simulink model "VFDnow"  (R2025b)
settings: Solver=VariableStepAuto  StartTime=0.0  StopTime=10  RelTol=1e-3
libraries: ee_lib x17, nesl_utility x12, fl_lib x10, dspstat3 x3, eePwmGeneratorTwoLevel x1, eeSinGeneratorThreePhase x1, simulink x1
settings Model: Creator=Administrator  LastModifiedBy=Nandana
settings SolverCC: AlgebraicLoopSolver=TrustRegion
settings DebuggingCC: UnconnectedInputMsg=warning  UnconnectedOutputMsg=warning  UnconnectedLineMsg=warning
settings ModelReferenceCC: EnableRefExpFcnMdlSchedulingChecks=on
settings SFSimCC: CustomCodeUndefinedFunction=UseInterfaceOnly
settings RTWCC: GPUComputeCapability=3.5  DLArmComputeVersion=19.05

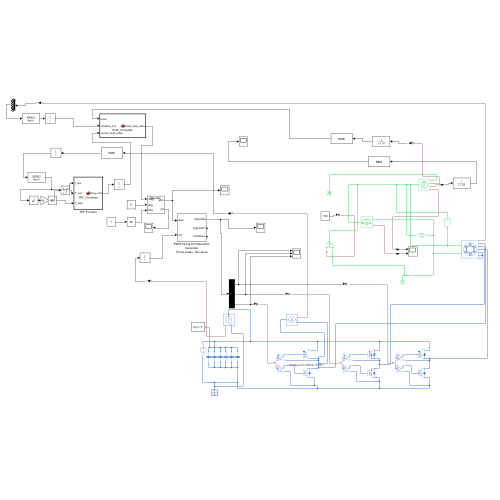
[thumbnail: Simulink's stored preview of the top-level diagram]
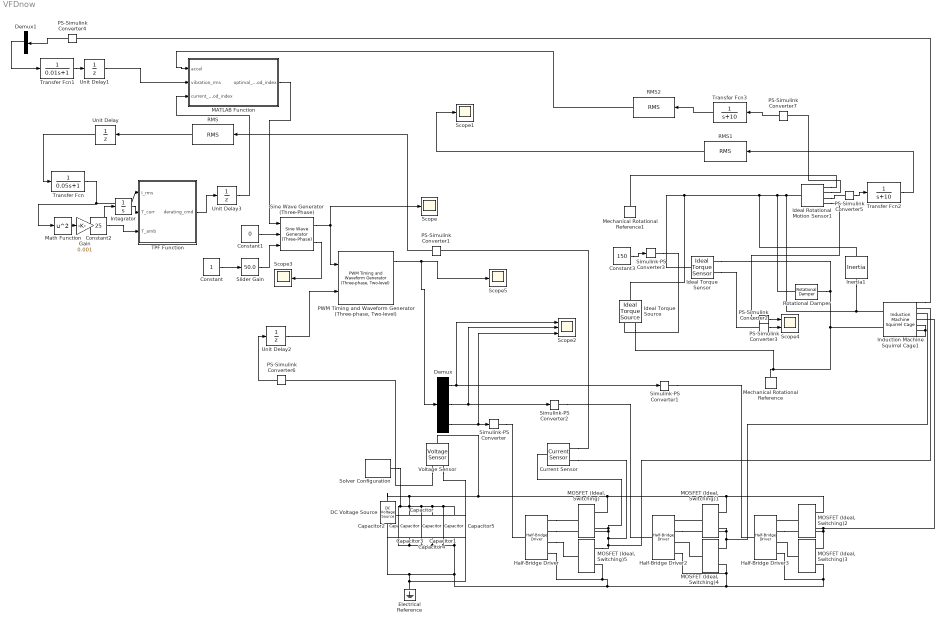
== system VFDnow ==
  Capacitor{,1..5} (6 alike) : ee_lib/Passive/Capacitor  cap_option=ee.enum.passive.capacitor.capOption.const  c=550e-6 F  Cvec=[1e-05, 1e-06] F  Vvec=[0, 10] V  CV_table_symmetry=ee.enum.passive.capacitor.tableSymmetry.yes  f_vec=[1, 10] kHz  DFext_vec=[.8, 1.2]  enable_C_tol=ee.enum.toleranceApplication.none  averaging_period=0 s  C_tol=5  tol_distribution=ee.enum.toleranceDistribution.uniform  nSigma=4  r=1 Ohm  g=0 1/Ohm  enable_operating_limits=ee.enum.enable.no  operating_limit_action=ee.enum.passive.reportOpLim.warn  max_working_voltage_range=[-25, 25] V  power_rating=1 W  maxTemperature=85 degC  thermalEnable=false  thermalMass=1 J/K  i_specify=off  i_priority=None  i=0 A  i_nominal_specify=off  i_nominal_value=1  i_nominal_unit=A  v_specify=on  v_priority=None  v=565 V  v_nominal_specify=off  v_nominal_value=1  v_nominal_unit=V  vc_specify=off  vc_priority=High  vc=0 V  vc_nominal_specify=off  vc_nominal_value=1  vc_nominal_unit=V  T_specify=off  T_priority=None  T=298.15 K  T_nominal_specify=off  T_nominal_value=1  T_nominal_unit=K
  Constant : Constant  SampleTime=1e-6
  Constant1 : Constant  Value=0  SampleTime=1e-6
  Constant2 : Constant  Value=25  SampleTime=1e-6
  Constant3 : Constant  Value=150  SampleTime=1e-6
  Current Sensor : fl_lib/Electrical/Electrical Sensors/Current Sensor
  DC Voltage Source : ee_lib/Additional Components/SPICE Sources/DC Voltage Source  DC=650 V
  Demux : Demux  Outputs=3
  Demux1 : Demux  Outputs=8
  Electrical Reference : fl_lib/Electrical/Electrical Elements/Electrical Reference
  Gain : Gain  Gain=0.001
  Half-Bridge Driver : ee_lib/Semiconductors & Converters/Half-Bridge Driver  port_option=ee.enum.controlport.ps  uHigh=2.0 V  uLow=0.8 V  uHighValue=0.7  uLowValue=0.3  vHigh=15 V  vLow=0 V  tpLH=50 ns  tdLH=100 ns  tpHL=50 ns  tdHL=100 ns  parameterization=ee.enum.semiconductors.gateDriverParam.outputImpedance  rHigh=2 Ohm  rLow=2 Ohm  tRise=20 ns  tFall=20 ns  cLoad=10 nF  ZonTime_specify=off  ZonTime_priority=None  ZonTime=0 s  ZoffTime_specify=off  ZoffTime_priority=None  ZoffTime=0 s  power_dissipated_high_side_specify=off  power_dissipated_high_side_priority=None  power_dissipated_high_side=0 W  power_dissipated_high_side_nominal_specify=off  power_dissipated_high_side_nominal_value=1  power_dissipated_high_side_nominal_unit=W  power_dissipated_low_side_specify=off  power_dissipated_low_side_priority=None  power_dissipated_low_side=0 W  power_dissipated_low_side_nominal_specify=off  power_dissipated_low_side_nominal_value=1  power_dissipated_low_side_nominal_unit=W
      settings: InternalSimscapePortConfiguration="{\"Bottom\":[],\"Left\":[{\"id\":\"u\",\"label\":\"u\",\"type\":\"input\"}],\"Right\":[{\"id\":\"HO\",\"label\":\"HO\",\"type\":\"foundation.electrical.electrical\"},{\"id\":\"HS\",\"label\":\"HS\",\"type\":\"foundation.electrical.electrical\"},{\"id\":\"LO\",\"label\":\"LO\",\"type\":\"foundation.electrical.electrical\"},{\"id\":\"LS\",\"label\":\"LS\",\"type\":\"foundation.electrical.electrical\"}],\"Top\":[]}"
  Half-Bridge Driver2 : ee_lib/Semiconductors & Converters/Half-Bridge Driver  port_option=ee.enum.controlport.ps  uHigh=2.0 V  uLow=0.8 V  uHighValue=0.7  uLowValue=0.3  vHigh=15 V  vLow=0 V  tpLH=50 ns  tdLH=100 ns  tpHL=50 ns  tdHL=100 ns  parameterization=ee.enum.semiconductors.gateDriverParam.outputImpedance  rHigh=2 Ohm  rLow=2 Ohm  tRise=20 ns  tFall=20 ns  cLoad=10 nF  ZonTime_specify=off  ZonTime_priority=None  ZonTime=0 s  ZoffTime_specify=off  ZoffTime_priority=None  ZoffTime=0 s  power_dissipated_high_side_specify=off  power_dissipated_high_side_priority=None  power_dissipated_high_side=0 W  power_dissipated_high_side_nominal_specify=off  power_dissipated_high_side_nominal_value=1  power_dissipated_high_side_nominal_unit=W  power_dissipated_low_side_specify=off  power_dissipated_low_side_priority=None  power_dissipated_low_side=0 W  power_dissipated_low_side_nominal_specify=off  power_dissipated_low_side_nominal_value=1  power_dissipated_low_side_nominal_unit=W
      settings: InternalSimscapePortConfiguration="{\"Bottom\":[],\"Left\":[{\"id\":\"u\",\"label\":\"u\",\"type\":\"input\"}],\"Right\":[{\"id\":\"HO\",\"label\":\"HO\",\"type\":\"foundation.electrical.electrical\"},{\"id\":\"HS\",\"label\":\"HS\",\"type\":\"foundation.electrical.electrical\"},{\"id\":\"LO\",\"label\":\"LO\",\"type\":\"foundation.electrical.electrical\"},{\"id\":\"LS\",\"label\":\"LS\",\"type\":\"foundation.electrical.electrical\"}],\"Top\":[]}"
  Half-Bridge Driver3 : ee_lib/Semiconductors & Converters/Half-Bridge Driver  port_option=ee.enum.controlport.ps  uHigh=2.0 V  uLow=0.8 V  uHighValue=0.7  uLowValue=0.3  vHigh=15 V  vLow=0 V  tpLH=50 ns  tdLH=100 ns  tpHL=50 ns  tdHL=100 ns  parameterization=ee.enum.semiconductors.gateDriverParam.outputImpedance  rHigh=2 Ohm  rLow=2 Ohm  tRise=20 ns  tFall=20 ns  cLoad=10 nF  ZonTime_specify=off  ZonTime_priority=None  ZonTime=0 s  ZoffTime_specify=off  ZoffTime_priority=None  ZoffTime=0 s  power_dissipated_high_side_specify=off  power_dissipated_high_side_priority=None  power_dissipated_high_side=0 W  power_dissipated_high_side_nominal_specify=off  power_dissipated_high_side_nominal_value=1  power_dissipated_high_side_nominal_unit=W  power_dissipated_low_side_specify=off  power_dissipated_low_side_priority=None  power_dissipated_low_side=0 W  power_dissipated_low_side_nominal_specify=off  power_dissipated_low_side_nominal_value=1  power_dissipated_low_side_nominal_unit=W
      settings: InternalSimscapePortConfiguration="{\"Bottom\":[],\"Left\":[{\"id\":\"u\",\"label\":\"u\",\"type\":\"input\"}],\"Right\":[{\"id\":\"HO\",\"label\":\"HO\",\"type\":\"foundation.electrical.electrical\"},{\"id\":\"HS\",\"label\":\"HS\",\"type\":\"foundation.electrical.electrical\"},{\"id\":\"LO\",\"label\":\"LO\",\"type\":\"foundation.electrical.electrical\"},{\"id\":\"LS\",\"label\":\"LS\",\"type\":\"foundation.electrical.electrical\"}],\"Top\":[]}"
  Ideal Rotational Motion Sensor1 : fl_lib/Mechanical/Mechanical Sensors/Ideal Rotational Motion Sensor  reference=foundation.enum.MeasurementReference.difference  acceleration_port=true  velocity_port=true  position_port=true  wrap_angle=false  offset=0 rad
      settings: InternalSimscapePortConfiguration="{\"Bottom\":[],\"Left\":[{\"id\":\"R\",\"label\":\"R\",\"type\":\"foundation.mechanical.rotational.rotational\"}],\"Right\":[{\"id\":\"C\",\"label\":\"C\",\"type\":\"foundation.mechanical.rotational.rotational\"},{\"id\":\"alpha\",\"label\":\"α\",\"type\":\"output\"},{\"id\":\"W\",\"label\":\"W\",\"type\":\"output\"},{\"id\":\"A\",\"label\":\"A\",\"type\":\"output\"}],\"Top\":[]}"
  Ideal Torque Sensor : fl_lib/Mechanical/Mechanical Sensors/Ideal Torque Sensor
  Ideal Torque Source : fl_lib/Mechanical/Mechanical Sources/Ideal Torque Source
  Induction Machine Squirrel Cage1 : ee_lib/Electromechanical/Asynchronous/Induction Machine Squirrel Cage  port_option=ee.enum.threePhasePort.expanded  SRated=15e3 A*V  VRated=220 V  FRated=60 Hz  nPolePairs=1  param_unit=ee.enum.unit.si  squirrel_cage=ee.enum.squirrelcage.Single  zero_sequence=ee.enum.park.zerosequence.include  initialization_option=ee.enum.asm.initialization.fluxvariables  Rs=0.25 Ohm  Xls=0.4 Ohm  pu_Rs=0.0258  pu_Lls=0.0413  Rrd=0.14 Ohm  Xlrd=0.41 Ohm  pu_Rrd=0.0145  pu_Llrd=0.0424  Rrd1=0.28 Ohm  Xlrd1=0.82 Ohm  Rrd2=0.28 Ohm  Xlrd2=0.82 Ohm  pu_Rrd1=0.0290  pu_Llrd1=0.0848  pu_Rrd2=0.0290  pu_Llrd2=0.0848  Xm=17 Ohm  pu_Lm=1.7562  X0=0.4 Ohm  pu_L0=0.0413  saturation_option=ee.enum.saturation.exclude  saturation_i=[0, 4, 9, 18, 25, 34, 50, 68, 95, 120] A  saturation_v=[0, 88, 154, 198, 220, 242, 264, 286, 308, 327] V  pu_saturation_i=[0, .176, .396, .792, 1.1, 1.496, 2.2, 2.992, 4.18, 5.28]  pu_saturation_v=[0, .4, .7, .9, 1, 1.1, 1.2, 1.3, 1.4, 1.4864]  connection_option=ee.enum.Connection.delta  angular_position_specify=off  angular_position_priority=None  angular_position=0 deg  angular_position_nominal_specify=off  angular_position_nominal_value=1  angular_position_nominal_unit=deg  pu_psids_specify=off  pu_psids_priority=None  pu_psids=0  pu_psids_nominal_specify=off  pu_psids_nominal_value=1  pu_psids_nominal_unit=1  pu_psiqs_specify=off  pu_psiqs_priority=None  pu_psiqs=0  pu_psiqs_nominal_specify=off  pu_psiqs_nominal_value=1  pu_psiqs_nominal_unit=1  pu_psi0s_specify=off  pu_psi0s_priority=None  pu_psi0s=0  pu_psi0s_nominal_specify=off  pu_psi0s_nominal_value=1  pu_psi0s_nominal_unit=1  pu_psidr_specify=off  pu_psidr_priority=None  pu_psidr=0  pu_psidr_nominal_specify=off  pu_psidr_nominal_value=1  pu_psidr_nominal_unit=1  pu_psiqr_specify=off  pu_psiqr_priority=None  pu_psiqr=0  pu_psiqr_nominal_specify=off  pu_psiqr_nominal_value=1  pu_psiqr_nominal_unit=1  pu_psidr1_specify=off  pu_psidr1_priority=None  pu_psidr1=0  pu_psidr1_nominal_specify=off  pu_psidr1_nominal_value=1  pu_psidr1_nominal_unit=1  pu_psiqr1_specify=off  pu_psiqr1_priority=None  pu_psiqr1=0  pu_psiqr1_nominal_specify=off  pu_psiqr1_nominal_value=1  pu_psiqr1_nominal_unit=1  pu_psidr2_specify=off  pu_psidr2_priority=None  pu_psidr2=0  pu_psidr2_nominal_specify=off  pu_psidr2_nominal_value=1  pu_psidr2_nominal_unit=1  pu_psiqr2_specify=off  pu_psiqr2_priority=None  pu_psiqr2=0  pu_psiqr2_nominal_specify=off  pu_psiqr2_nominal_value=1  pu_psiqr2_nominal_unit=1  psids_specify=off  psids_priority=None  psids=0 Wb  psids_nominal_specify=off  psids_nominal_value=1  psids_nominal_unit=Wb  psiqs_specify=off  psiqs_priority=None  psiqs=0 Wb  psiqs_nominal_specify=off  psiqs_nominal_value=1  psiqs_nominal_unit=Wb  psi0s_specify=off  psi0s_priority=None  psi0s=0 Wb  psi0s_nominal_specify=off  psi0s_nominal_value=1  psi0s_nominal_unit=Wb  psidr_specify=off  psidr_priority=None  psidr=0 Wb  psidr_nominal_specify=off  psidr_nominal_value=1  psidr_nominal_unit=Wb  psiqr_specify=off  psiqr_priority=None  psiqr=0 Wb  psiqr_nominal_specify=off  psiqr_nominal_value=1  psiqr_nominal_unit=Wb  psidr1_specify=off  psidr1_priority=None  psidr1=0 Wb  psidr1_nominal_specify=off  psidr1_nominal_value=1  psidr1_nominal_unit=Wb  psiqr1_specify=off  psiqr1_priority=None  psiqr1=0 Wb  psiqr1_nominal_specify=off  psiqr1_nominal_value=1  psiqr1_nominal_unit=Wb  psidr2_specify=off  psidr2_priority=None  psidr2=0 Wb  psidr2_nominal_specify=off  psidr2_nominal_value=1  psidr2_nominal_unit=Wb  psiqr2_specify=off  psiqr2_priority=None  psiqr2=0 Wb  psiqr2_nominal_specify=off  psiqr2_nominal_value=1  psiqr2_nominal_unit=Wb  slip_specify=off  slip_priority=None  slip=0  slip_nominal_specify=off  slip_nominal_value=1  slip_nominal_unit=1  real_power_generated_specify=off  real_power_generated_priority=None  real_power_generated=0 W  real_power_generated_nominal_specify=off  real_power_generated_nominal_value=1  real_power_generated_nominal_unit=W  mechanical_power_consumed_specify=off  mechanical_power_consumed_priority=None  mechanical_power_consumed=0 W  mechanical_power_consumed_nominal_specify=off  mechanical_power_consumed_nominal_value=1  mechanical_power_consumed_nominal_unit=W  Tmeas=298.15 K  alpha=3.93e-3 1/K  alpha_cage=4.4e-3 1/K  stator_thermal_mass=100 J/K  rotor_thermal_mass=200 J/K  temperatureA_specify=off  temperatureA_priority=High  temperatureA=25 degC  temperatureA_nominal_specify=off  temperatureA_nominal_value=1  temperatureA_nominal_unit=degC  temperatureB_specify=off  temperatureB_priority=High  temperatureB=25 degC  temperatureB_nominal_specify=off  temperatureB_nominal_value=1  temperatureB_nominal_unit=degC  temperatureC_specify=off  temperatureC_priority=High  temperatureC=25 degC  temperatureC_nominal_specify=off  temperatureC_nominal_value=1  temperatureC_nominal_unit=degC  temperatureR_specify=off  temperatureR_priority=High  temperatureR=25 degC  temperatureR_nominal_specify=off  temperatureR_nominal_value=1  temperatureR_nominal_unit=degC
      settings: InternalSimscapePortConfiguration="{\"Bottom\":[],\"Left\":[{\"id\":\"R\",\"label\":\"R\",\"type\":\"foundation.mechanical.rotational.rotational\"},{\"id\":\"C\",\"label\":\"C\",\"type\":\"foundation.mechanical.rotational.rotational\"}],\"Right\":[{\"id\":\"pu_output\",\"label\":\"pu\",\"type\":\"output\"},{\"id\":\"a1\",\"label\":\"a1\",\"type\":\"foundation.electrical.electrical\"},{\"id\":\"b1\",\"label\":\"b1\",\"type\":\"foundation.electrical.electrical\"},{\"id\":\"c1\",\"label\":\"c1\",\"type\":\"foundation.electrical.electrical\"},{\"id\":\"a2\",\"label\":\"a2\",\"type\":\"foundation.electrical.electrical\"},{\"id\":\"b2\",\"label\":\"b2\",\"type\":\"foundation.electrical.electrical\"},{\"id\":\"c2\",\"label\":\"c2\",\"type\":\"foundation.electrical.electrical\"}],\"Top\":[]}"
  Inertia1 : fl_lib/Mechanical/Rotational Elements/Inertia  inertia=1.8 kg*m^2  num_ports=foundation.enum.numPorts2.two  w_specify=off  w_priority=High  w=0 rad/s  w_nominal_specify=off  w_nominal_value=1  w_nominal_unit=rad/s  t_specify=off  t_priority=None  t=0 N*m  t_nominal_specify=off  t_nominal_value=1  t_nominal_unit=N*m
      settings: InternalSimscapePortConfiguration="{\"Bottom\":[],\"Left\":[{\"id\":\"I\",\"label\":\"\",\"type\":\"foundation.mechanical.rotational.rotational\"}],\"Right\":[{\"id\":\"J\",\"label\":\"\",\"type\":\"foundation.mechanical.rotational.rotational\"}],\"Top\":[]}"
  Integrator : Integrator  InitialCondition=25  LimitOutput=on  UpperSaturationLimit=100  LowerSaturationLimit=25
  MATLAB Function : MATLAB Function  TreatAsAtomicUnit=on
  "MOSFET (Ideal, Switching)" : ee_lib/Semiconductors & Converters/MOSFET (Ideal, Switching)  PartSpecification="{\"CollectionId\":\"SimscapeElectrical\",\"CollectionVersion\":\"1.0.0\",\"DatasetId\":\"Wolfspeed|C3M0021120K1|\",\"DisplayName\":\"Wolfspeed:C3M0021120K1\"}"  port_option=ee.enum.controlport.elec  Rds=0.021 % Datasheet derived Ohm  Goff=8.33333333333333e-10 % Datasheet derived S  Vth=2.9 % Wolfspeed XML derived V  diode_param=ee.enum.converters.protectiondiode.nodynamics  diode_Vf=2.47 % Datasheet derived V  diode_Ron=0.012 % Wolfspeed XML derived Ohm  diode_Goff=1e-05 % Library default S  diode_C=50e-9 % Parameter not set F  diode_iRM=-235 % Parameter not set A  diode_iF=300 % Parameter not set A  diode_idot=-50 % Parameter not set A/us  diode_trr_param=ee.enum.converters.diodeReverseParam.trr_factor  diode_trr_factor=3 % Parameter not set  diode_trr=15 % Parameter not set us  diode_Qrr=1500 % Parameter not set s*uA  ids_specify=on  ids_priority=None  ids=0 A  ids_nominal_specify=on  ids_nominal_value=1  ids_nominal_unit=A  vds_specify=on  vds_priority=None  vds=0 V  vds_nominal_specify=on  vds_nominal_value=1  vds_nominal_unit=V  vgs_specify=off  vgs_priority=None  vgs=0 V  vgs_nominal_specify=off  vgs_nominal_value=1  vgs_nominal_unit=V  thermal_loss_option=ee.enum.converters.thermalLossOption.tabulated2d  Von_data=[-4.27389 -4.02367 -3.77256 -3.51776 -3.26306 -3.00223 -2.73772 -2.46956 -2.19212 -1.90551 -1.60743 -1.29443 -0.962781 -0.606415 -0.31632 -0.214648 -0.108889 -0.0455276 -0.0237427 0 0.0228239 0.0433363 0.106503 0.214663 0.323026 0.662263 1.13841 1.64037 2.16245 2.70962 3.28471 3.8982 4.56044 5.2802 6.07016 6.93522;-5.18634 -4.76738 -4.4029 -4.06633 -3.72922 -3.39492 -3.05953 -2.72304 -2.38461 -2.04123 -1.69306 -1.33736 -0.97293 -0.595048 -0.302935 -0.206772 -0.104318 -0.0429045 -0.0221598 0 0.0232804 0.0430606 0.104009 0.206365 0.308279 0.6242 1.06384 1.5255 2.0111 2.52481 3.07168 3.65807 4.29107 4.98079 5.73956 6.58181;-8.32654 -7.93499 -7.51349 -7.06183 -6.57553 -6.05033 -5.48279 -4.87921 -4.25441 -3.61939 -2.97325 -2.32248 -1.66914 -1.01052 -0.510784 -0.341428 -0.172389 -0.0707504 -0.0361764 0 0.0365721 0.0707068 0.173457 0.346572 0.520136 1.04549 1.76862 2.5225 3.31582 4.16389 5.07499 6.06793 7.16531 8.3916 9.78437 11.3885;-9.1592 -8.72849 -8.26484 -7.76802 -7.23309 -6.65536 -6.03107 -5.36713 -4.67985 -3.98133 -3.27058 -2.55473 -1.83605 -1.11158 -0.561862 -0.375571 -0.189628 -0.0778255 -0.039794 0 0.0402293 0.0777775 0.190803 0.381229 0.57215 1.15004 1.94548 2.77475 3.6474 4.58028 5.58249 6.67472 7.88184 9.23076 10.7628 12.5274] % Wolfspeed XML derived V  Tj=[-55 25 175 900] % Wolfspeed XML derived degC  Iout_data=[-290 -270 -250 -230 -210 -190 -170 -150 -130 -110 -90 -70 -50 -30 -15 -10 -5 -2 -1 0 1 2 5 10 15 30 50 70 90 110 130 150 170 190 210 230] % Wolfspeed XML derived A  Eon_data=[0 0.00041745 0.0006665 0.0009583 0.0013038 0.0016836 0.0021011 0.0025367 0.0029961;0 0.00043908 0.00072163 0.0010599 0.001457 0.0018976 0.0023654 0.0028532 0.0033508;0 0.00049099 0.00084535 0.0012573 0.0017203 0.0022304 0.0027638 0.0032706 0.0036897;0 0.0005622 0.00099378 0.0014717 0.0019935 0.0025368 0.0030168 0.0033994 0.0036872;0 0.00061842 0.0010932 0.0016189 0.0021929 0.0027904 0.0033184 0.0037393 0.0040559] % Wolfspeed XML derived J  Eoff_data=[0 7.5223e-05 0.00013186 0.0002269 0.00034998 0.00048869 0.00064891 0.00082419 0.0010195;0 8.254e-05 0.000147 0.00025079 0.00037991 0.00052991 0.00069891 0.00088752 0.0010918;0 7.4201e-05 0.00015201 0.00026409 0.0004049 0.00056157 0.00074296 0.00093905 0.0011553;0 8.0776e-05 0.00015818 0.00028047 0.0004289 0.00059195 0.00078795 0.00099015 0.0012074;0 8.8853e-05 0.000174 0.00030852 0.00047179 0.00065115 0.00086674 0.0010892 0.0013281] % Wolfspeed XML derived J  Eon_data_3D=reshape([0;0;0;0;0;0;0;0;0;0;0;0;0;0;0;0;0;0;0;0;0;0;0;0;0;0;0;0;0;0;0;0;0;0;0;0;0;0;0;0;0;0;0;0;0;0;0;0;0;0;0;0;0;0;0;0;0;0;0;0;0;0;0;0;0;0;0;0;0;0;0;0;0;0;0;0;0;0;0;0;0;0;0;0;0;0;0;0;0;0;0;0;0;0;0;0.0002788;0.0002932;0.00032775;0.00037518;0.0004127;0.00043572;0.00047148;0.00055198;0.00064879;0.00071367;0.0006243;0.0006901;0.00081857;0.00095848;0.0010543;0.00085437;0.00095468;0.0011272;0.0013064;0.0014371;0.0010984;0.0012379;0.0014553;0.0016574;0.0018231;0.0013696;0.0015419;0.0018028;0.0019726;0.0021698;0.0016665;0.0018748;0.0021525;0.0022422;0.0024665;0.0019653;0.0021993;0.0024309;0.0024363;0.0026799;0;0;0;0;0;0.00041745;0.00043908;0.00049099;0.0005622;0.00061842;0.0006665;0.00072163;0.00084535;0.00099378;0.0010932;0.0009583;0.0010599;0.0012573;0.0014717;0.0016189;0.0013038;0.001457;0.0017203;0.0019935;0.0021929;0.0016836;0.0018976;0.0022304;0.0025368;0.0027904;0.0021011;0.0023654;0.0027638;0.0030168;0.0033184;0.0025367;0.0028532;0.0032706;0.0033994;0.0037393;0.0029961;0.0033508;0.0036897;0.0036872;0.0040559],[5 9 4]) % Wolfspeed XML derived J  Eoff_data_3D=reshape([0;0;0;0;0;0;0;0;0;0;0;0;0;0;0;0;0;0;0;0;0;0;0;0;0;0;0;0;0;0;0;0;0;0;0;0;0;0;0;0;0;0;0;0;0;0;0;0;0;0;0;0;0;0;0;0;0;0;0;0;0;0;0;0;0;0;0;0;0;0;0;0;0;0;0;0;0;0;0;0;0;0;0;0;0;0;0;0;0;0;0;0;0;0;0;4.6339e-05;5.0834e-05;4.5637e-05;4.9715e-05;5.4686e-05;8.9796e-05;0.00010011;0.00010338;0.00010758;0.00011833;0.00015204;0.00016814;0.00017697;0.00018789;0.00020668;0.00024257;0.00026333;0.00028065;0.0002973;0.00032703;0.00034178;0.00037067;0.00039283;0.00041406;0.00045547;0.00045429;0.00048937;0.00052024;0.00055174;0.00060691;0.0005861;0.00063122;0.00066795;0.00070456;0.00077502;0.00072968;0.00078189;0.00082724;0.00086523;0.00095175;0;0;0;0;0;7.5223e-05;8.254e-05;7.4201e-05;8.0776e-05;8.8853e-05;0.00013186;0.000147;0.00015201;0.00015818;0.000174;0.0002269;0.00025079;0.00026409;0.00028047;0.00030852;0.00034998;0.00037991;0.0004049;0.0004289;0.00047179;0.00048869;0.00052991;0.00056157;0.00059195;0.00065115;0.00064891;0.00069891;0.00074296;0.00078795;0.00086674;0.00082419;0.00088752;0.00093905;0.00099015;0.0010892;0.0010195;0.0010918;0.0011553;0.0012074;0.0013281],[5 9 4]) % Wolfspeed XML derived J  Tj_loss=[25 75 125 175 900] % Wolfspeed XML derived degC  Iout_data_loss=[0 16.48625 31.86563 46.89437 62.43531 76.75938 91.2175 105.2391 119.1231] % Wolfspeed XML derived A  tabulateWithVds=true  Vds_loss=[-100 0 600 800] % Wolfspeed XML derived V  Eon_scalar=22.86e-3 % Parameter not set J  Eoff_scalar=17.14e-3 % Parameter not set J  Voff=300 % Parameter not set V  Iout_scalar=600 % Parameter not set A  useCurrentFromPreviousCycle=false % Parameter not set  useVoltageFromPreviousCycle=false % Parameter not set  diodeModelType=ee.enum.converters.diodeModelType.tabulated  diodeTableType=ee.enum.diode.tableType.VfMat  diode_ReverseIVType=ee.enum.diode.diodeReverseIV.constant  diode_IfMat=[.07, .12, .19, 1.75, 4.24, 7.32, 11.2; .16, .3, .72, 2.14, 4.02, 6.35, 9.12] % Parameter not set A  diode_VfMat=[0 3.4539 3.7122 4.1778 4.6574 5.0077 5.7507 6.4353 6.9636 7.4039 7.7872 8.1335 8.4486 8.7404 9.0146 9.2743 9.5227 9.7598 9.9906;0 3.0632 3.2597 3.6226 4.0058 4.2921 4.9319 5.5601 6.0709 6.512 6.909 7.2724 7.6085 7.9244 8.2241 8.5101 8.7827 9.0425 9.2923;0 2.6447 2.8328 3.1828 3.5428 3.8081 4.3889 4.9604 5.4274 5.8323 6.1991 6.5353 6.8489 7.1419 7.4196 7.6847 7.9366 8.1816 8.4159;0 2.1158 2.2663 2.5462 2.8343 3.0464 3.5111 3.9683 4.3419 4.6658 4.9593 5.2283 5.4792 5.7135 5.9357 6.1478 6.3493 6.5453 6.7327] % Wolfspeed XML derived V  diode_TjVec=[-55 25 175 900] % Wolfspeed XML derived degC  diode_VfVec=[.5, .7, .9, 1.3, 1.7, 2.1, 2.5] % Parameter not set V  diode_IfVec=[0 1 2 5 10 15 30 50 70 90 110 130 150 170 190 210 230 250 270] % Wolfspeed XML derived A  diode_IrMat=[1e-06, 2e-06, 5e-06, 1e-05, 2.5e-05, 5e-05, .0001; 2e-06, 5e-06, 1e-05, 4e-05, 8e-05, .0002, .0005] % Parameter not set A  diode_VrMat=[10, 100, 200, 250, 300, 325, 350; 10, 70, 160, 220, 270, 300, 320] % Parameter not set V  diode_VrVec=[10, 20, 40, 50, 70, 80, 100] % Parameter not set V  diode_IrVec=[1e-06, 2e-06, 5e-06, 1e-05, 2e-05, 5e-05, .0001] % Parameter not set A  diode_Vr=-600 % Parameter not set V  diode_Ls=150 % Parameter not set nH  diode_Erec=0.03 % Parameter not set J  diode_rec_loss_model=ee.enum.diode.reverseRecoveryModel.tabulated2d  diode_ErecVal=0 % Parameter not set J  diode_scaleWithIandV=true % Parameter not set  diode_ErecMat=[0 0;0 0] % Wolfspeed XML derived J  diode_TjrecVec=[25 35] % Wolfspeed XML derived degC  diode_IfrecVec=[0 10] % Wolfspeed XML derived A  diode_IrecVal=10 % Parameter not set A  diode_VrecVal=10 % Wolfspeed XML derived V  diode_tFilter=1 / 1000 / 100 % Parameter not set s  separateThermalPortForDiode=true  thermal_network_parameterization=ee.enum.thermalNetworkTopology.cauer  Rth=[.03, .2] % Parameter not set K/W  Rth_Cauer=[0.040655 0.093503 0.046885 0.094584] % Wolfspeed XML derived K/W  Rth_Foster=[.08, .14, .22, .16] % Parameter not set K/W  thermal_mass_parameterization=ee.enum.thermalNetwork.thermalmass  thermal_mass=[3, 25] % Parameter not set J/K  thermal_mass_Cauer=[0.0029508 0.016009 0.049724 0.13401] % Wolfspeed XML derived J/K  thermal_mass_Foster=[.001, .005, .05, .5] % Parameter not set J/K  thermal_time_constant=[.1, 5] % Parameter not set s  thermal_time_constant_Cauer=[.1, 1, 5] % Parameter not set s  thermal_time_constant_Foster=[7e-05, .0007, .01, .08] % Parameter not set s  thermal_mass_initial_temperatures=[25, 25] % Parameter not set degC  thermal_mass_initial_temperatures_Cauer=[25 25 25 25] % Wolfspeed XML derived degC  junction_thermal_mass=0.1 % Parameter not set J/K  Tvec_initial_Foster=[25, 25, 25, 25] % Parameter not set degC  RthDiode=[.03, .2] % Parameter not set K/W  RthCauerDiode=[0.040655 0.093503 0.046885 0.094584] % Wolfspeed XML derived K/W  RthFosterDiode=[.03, .2] % Parameter not set K/W  thermalMassDiode=[3, 25] % Parameter not set J/K  thermalMassCauerDiode=[0.0029508 0.016009 0.049724 0.13401] % Wolfspeed XML derived J/K  thermalMassFosterDiode=[33, 50] % Parameter not set J/K  thermalTauDiode=[.1, 5] % Parameter not set s  thermalTauCauerDiode=[.1, 1, 5] % Parameter not set s  thermalTauFosterDiode=[1, 10] % Parameter not set s  thermalMassInitTempDiode=[25, 25] % Parameter not set degC  thermalMassInitTempCauerDiode=[25 25 25 25] % Wolfspeed XML derived degC  junctionthermalMassDiode=0.1 % Parameter not set J/K  TVecInitialFosterDiode=[25, 25, 25, 25] % Parameter not set degC  no_thermal_network=0 % Parameter not set  mosfet_junction_temperature_specify=off  mosfet_junction_temperature_priority=None  mosfet_junction_temperature=25 degC  mosfet_junction_temperature_nominal_specify=off  mosfet_junction_temperature_nominal_value=1  mosfet_junction_temperature_nominal_unit=degC  diode_junction_temperature_specify=off  diode_junction_temperature_priority=None  diode_junction_temperature=25 degC  diode_junction_temperature_nominal_specify=off  diode_junction_temperature_nominal_value=1  diode_junction_temperature_nominal_unit=degC  Qj_specify=off  Qj_priority=None  Qj=0 W  Qj_nominal_specify=off  Qj_nominal_value=1  Qj_nominal_unit=W  accumulatedSwitchingLosses_specify=off  accumulatedSwitchingLosses_priority=None  accumulatedSwitchingLosses=0 J
      settings: AttributesFormatString=Wolfspeed:C3M0021120K1  InternalSimscapePortConfiguration="{\"Bottom\":[],\"Left\":[{\"id\":\"G_elec\",\"label\":\"\",\"type\":\"foundation.electrical.electrical\"}],\"Right\":[{\"id\":\"D\",\"label\":\"\",\"type\":\"foundation.electrical.electrical\"},{\"id\":\"S\",\"label\":\"\",\"type\":\"foundation.electrical.electrical\"}],\"Top\":[]}"
  MOSFET (Ideal, Switching){1..5} (5 alike) : ee_lib/Semiconductors & Converters/MOSFET (Ideal, Switching)  port_option=ee.enum.controlport.elec  Rds=0.01 Ohm  Goff=1e-6 1/Ohm  Vth=2 V  diode_param=ee.enum.semiconductors.protectionDiode.nodynamics  diode_Vf=0.8 V  diode_Ron=0.001 Ohm  diode_Goff=1e-5 1/Ohm  diode_C=50e-9 F  diode_iRM=-235 A  diode_iF=300 A  diode_idot=-50 A/us  diode_trr_param=ee.enum.converters.diodeReverseParam.trr_factor  diode_trr_factor=3  diode_trr=15 us  diode_Qrr=1500 s*uA  ids_specify=off  ids_priority=None  ids=0 A  ids_nominal_specify=off  ids_nominal_value=1  ids_nominal_unit=A  vds_specify=off  vds_priority=None  vds=0 V  vds_nominal_specify=off  vds_nominal_value=1  vds_nominal_unit=V  vgs_specify=off  vgs_priority=None  vgs=0 V  vgs_nominal_specify=off  vgs_nominal_value=1  vgs_nominal_unit=V  thermal_loss_option=ee.enum.converters.thermalLossOption.constantvalues  Von_data=[0, 1.8, 3.2, 6, 10, 16; 0, 2, 5.5, 9.5, 15, 25] V  Tj=[298.15, 448.15] K  Iout_data=[0, 20, 40, 60, 80, 100] A  Eon_data=[0, 55.04, 124.57, 235.53, 362.12; 0, 71.25, 161.25, 304.88, 468.75] * 1e-6 J  Eoff_data=[0, 18, 30, 56.1, 76.5; 0, 22.5, 37.5, 70.13, 95.63] * 1e-6 J  Eon_data_3D=[zeros(2, 5, 3)] J  Eoff_data_3D=[zeros(2, 5, 3)] J  Tj_loss=[298.15, 448.15] K  Iout_data_loss=[0, 10, 20, 30, 40] A  tabulateWithVds=false  Vds_loss=[0, 150, 300] V  Eon_scalar=22.86e-3 J  Eoff_scalar=17.14e-3 J  Voff=300 V  Iout_scalar=600 A  useCurrentFromPreviousCycle=false  useVoltageFromPreviousCycle=false  diodeModelType=ee.enum.converters.diodeModelType.pwl  diodeTableType=ee.enum.diode.tableType.IfMat  diode_ReverseIVType=ee.enum.diode.diodeReverseIV.constant  diode_IfMat=[.07, .12, .19, 1.75, 4.24, 7.32, 11.2; .16, .3, .72, 2.14, 4.02, 6.35, 9.12] A  diode_VfMat=[.9, 1.15, 1.25, 1.5, 1.75, 2.17, 2.6, 2.85; .58, .68, .75, 1.1, 1.38, 1.77, 2.27, 2.7] V  diode_TjVec=[25, 125] degC  diode_VfVec=[.5, .7, .9, 1.3, 1.7, 2.1, 2.5] V  diode_IfVec=[.1, .2, .5, 1, 2, 4, 7, 10] A  diode_IrMat=[1e-06, 2e-06, 5e-06, 1e-05, 2.5e-05, 5e-05, .0001; 2e-06, 5e-06, 1e-05, 4e-05, 8e-05, .0002, .0005] A  diode_VrMat=[10, 100, 200, 250, 300, 325, 350; 10, 70, 160, 220, 270, 300, 320] V  diode_VrVec=[10, 20, 40, 50, 70, 80, 100] V  diode_IrVec=[1e-06, 2e-06, 5e-06, 1e-05, 2e-05, 5e-05, .0001] A  diode_Vr=-600 V  diode_Ls=150 nH  diode_Erec=0.03 J  diode_rec_loss_model=ee.enum.diode.reverseRecoveryModel.fixed  diode_ErecVal=0 J  diode_scaleWithIandV=true  diode_ErecMat=zeros(2, 3) J  diode_TjrecVec=[298.15, 398.15] K  diode_IfrecVec=[.1, 1, 10] A  diode_IrecVal=10 A  diode_VrecVal=10 V  diode_tFilter=1 / 1000 / 100 s  separateThermalPortForDiode=false  thermal_network_parameterization=ee.enum.thermalNetworkTopology.external  Rth=[.03, .2] K/W  Rth_Cauer=[.03, .1, .2] K/W  Rth_Foster=[.08, .14, .22, .16] K/W  thermal_mass_parameterization=ee.enum.thermalNetwork.timeconstant  thermal_mass=[3, 25] J/K  thermal_mass_Cauer=[3, 10, 25] J/K  thermal_mass_Foster=[.001, .005, .05, .5] J/K  thermal_time_constant=[.1, 5] s  thermal_time_constant_Cauer=[.1, 1, 5] s  thermal_time_constant_Foster=[7e-05, .0007, .01, .08] s  thermal_mass_initial_temperatures=[25, 25] degC  thermal_mass_initial_temperatures_Cauer=[25, 25, 25] degC  junction_thermal_mass=0.1 J/K  Tvec_initial_Foster=[25, 25, 25, 25] degC  RthDiode=[.03, .2] K/W  RthCauerDiode=[.03, .1, .2] K/W  RthFosterDiode=[.03, .2] K/W  thermalMassDiode=[3, 25] J/K  thermalMassCauerDiode=[3, 10, 25] J/K  thermalMassFosterDiode=[33, 50] J/K  thermalTauDiode=[.1, 5] s  thermalTauCauerDiode=[.1, 1, 5] s  thermalTauFosterDiode=[1, 10] s  thermalMassInitTempDiode=[25, 25] degC  thermalMassInitTempCauerDiode=[25, 25, 25] degC  junctionthermalMassDiode=0.1 J/K  TVecInitialFosterDiode=[25, 25, 25, 25] degC  no_thermal_network=0  mosfet_junction_temperature_specify=off  mosfet_junction_temperature_priority=None  mosfet_junction_temperature=25 degC  mosfet_junction_temperature_nominal_specify=off  mosfet_junction_temperature_nominal_value=1  mosfet_junction_temperature_nominal_unit=degC  diode_junction_temperature_specify=off  diode_junction_temperature_priority=None  diode_junction_temperature=25 degC  diode_junction_temperature_nominal_specify=off  diode_junction_temperature_nominal_value=1  diode_junction_temperature_nominal_unit=degC  Qj_specify=off  Qj_priority=None  Qj=0 W  Qj_nominal_specify=off  Qj_nominal_value=1  Qj_nominal_unit=W  accumulatedSwitchingLosses_specify=off  accumulatedSwitchingLosses_priority=None  accumulatedSwitchingLosses=0 J
      settings: InternalSimscapePortConfiguration="{\"Bottom\":[],\"Left\":[{\"id\":\"G_elec\",\"label\":\"\",\"type\":\"foundation.electrical.electrical\"}],\"Right\":[{\"id\":\"D\",\"label\":\"\",\"type\":\"foundation.electrical.electrical\"},{\"id\":\"S\",\"label\":\"\",\"type\":\"foundation.electrical.electrical\"}],\"Top\":[]}"
  Math Function : Math  Operator=square
  Mechanical Rotational Reference : fl_lib/Mechanical/Rotational Elements/Mechanical Rotational Reference
  Mechanical Rotational Reference1 : fl_lib/Mechanical/Rotational Elements/Mechanical Rotational Reference
  PS-Simulink Converter{1..2,4..7} (6 alike) : nesl_utility/PS-Simulink Converter  PhysicalDomain=network_engine_domain  SubClassName=ps_output  LeftPortType=input  RightPortType=output  PseudoPeriodic=off  Frequencies=[]  VectorFormat=inherit  Unit=inherit  AffineConversion=off
  PS-Simulink Converter3 : nesl_utility/PS-Simulink Converter  PhysicalDomain=network_engine_domain  SubClassName=ps_output  LeftPortType=input  RightPortType=output  PseudoPeriodic=off  Frequencies=[]  VectorFormat=inherit  Unit=rad  AffineConversion=off
  "PWM Timing and Waveform Generator (Three-phase, Two-level)" : eePwmGeneratorTwoLevel/PWM Timing and Waveform Generator (Three-phase, Two-level)  PWMMode=Continuous PWM (CPWM)  CPWMMode=SVM: space vector modulation  DPWMMode=60 DPWM (-30 degree shift): -30 degree shift from 60 DPWM  fsw=16000
      settings: SamplingMode=Natural
      settings: LibrarySourceBlock=|
      | ee_sl_lib/Pulse Width
      | Modulation/PWM Timing and Waveform
      | Generator
      | (Three-phase, Two-level)
  RMS : dspstat3/RMS  run=off  directionMode=Each column  dimension=1  InputProcessing=Columns as channels (frame based)  reset_popup=None
  RMS1 : dspstat3/RMS  run=off  directionMode=Each column  dimension=1  InputProcessing=Columns as channels (frame based)  reset_popup=None
  RMS2 : dspstat3/RMS  run=off  directionMode=Each column  dimension=1  InputProcessing=Columns as channels (frame based)  reset_popup=None
  Rotational Damper : fl_lib/Mechanical/Rotational Elements/Rotational Damper  D=0.05 N*m*s/rad  w_specify=off  w_priority=None  w=0 rad/s  w_nominal_specify=off  w_nominal_value=1  w_nominal_unit=rad/s  t_specify=off  t_priority=None  t=0 N*m  t_nominal_specify=off  t_nominal_value=1  t_nominal_unit=N*m
  Scope{,1,3,5} (4 alike) : Scope
      Scope settings: ActiveDisplayYMinimum=0.23817088996397734  ActiveDisplayYMaximum=0.25157848250419529
      Scope1 settings: ActiveDisplayYMinimum=-0.67417374525442053  ActiveDisplayYMaximum=1.0049836678211534
      Scope3 settings: ActiveDisplayYMinimum=-4.58577338507015  ActiveDisplayYMaximum=9.4544203181019419  DataLoggingVariableName=ScopeData3
      Scope5 settings: ActiveDisplayYMinimum=1.5573475654601123E-5  ActiveDisplayYMaximum=1.5676524345398877E-5  DataLoggingVariableName=ScopeData5
  Scope2 : Scope  NumInputPorts=3
      settings: ActiveDisplayYMinimum=1.559590351857362E-5  ActiveDisplayYMaximum=1.5647242039954659E-5  DataLoggingVariableName=ScopeData2
  Scope4 : Scope  NumInputPorts=2
      settings: ActiveDisplayYMinimum=-194.35610889768091  ActiveDisplayYMaximum=175.71484209304583  DataLoggingVariableName=ScopeData4
  Simulink-PS Converter{,1..3} (4 alike) : nesl_utility/Simulink-PS Converter  PhysicalDomain=network_engine_domain  SubClassName=ps_input  LeftPortType=input  RightPortType=output  PseudoPeriodic=off  Frequencies=[]  NoiseDistribution=none  NoiseParameters=[]  Unit=1  AffineConversion=off  FilteringAndDerivatives=provide  SimscapeFilterOrder=1  InputFilterTimeConstant=0.001  UdotUserProvided=0
  Sine Wave Generator (Three-Phase) : eeSinGeneratorThreePhase/Sine Wave Generator (Three-Phase)  Ts=1e-6
      settings: LibrarySourceBlock=|
      | ee_sl_lib/General Control/Sine Wave Generator
      | (Three-Phase)
  Slider Gain : simulink/Math Operations/Slider Gain  gain=50.0  low=0  high=100
  Solver Configuration : nesl_utility/Solver Configuration  PhysicalDomain=network_engine_domain  SubClassName=solver  LeftPortType=input  RightPortType=generic  Tones=[]  Harmonics=[]  SimulateNoise=off  Profile=off  UseLocalSampling=off  EnableSwitchedLinearOptims=on  FrequencyDomain=off  UseCCode=off  RelTol=0.001  AbsTol=0.001  MinStep=1e-09  ToWorkspace=off  RevertToSquareIcSolve=off  NumHomotopyIterations=100  PhasorMode=off  PhasorModeNumHarmonics=1  ConsistencySolver=NEWTON_XTOL_AFTER_FTOL  IndexReductionMethod=DerivativeReplacement  DoDC=off  ResidualTolerance=1e-09  ConsistencyTolSource=GLOBAL  ConsistencyAbsTol=0.001  ConsistencyRelTol=0.001  ConsistencyTolFactor=0.01  UseLocalSolver=on  LocalSolverChoice=NE_BACKWARD_EULER_ADVANCER  ResolveIndetEquations=on  FunctionEvalNumThread=1  LocalSolverSampleTime=1e-6  DoFixedCost=off  MaxNonlinIter=3  MaxModeIter=2  ComputeImpulses=off  ImpulseIterations=2  LinearAlgebra=Sparse  LinearAlgebraNumThread=0  EquationFormulation=NE_TIME_EF  DelaysMemoryBudget=1024  AutomaticFiltering=on  FilteringTimeConstant=0.001  PartitionStorageMethod=AS_NEEDED  PartitionMemoryBudget=1024  PartitionMethod=ROBUST  MultibodyUseLocalSolver=off  MultibodyLocalSolverChoice=ODE1  MultibodyLocalSolverSampleTime=0.001
  TPF Function : MATLAB Function  TreatAsAtomicUnit=on
  Transfer Fcn : TransferFcn  Denominator=[0.05 1]
  Transfer Fcn1 : TransferFcn  Denominator=[0.01 1]
  Transfer Fcn2 : TransferFcn  Denominator=[1 10]
  Transfer Fcn3 : TransferFcn  Denominator=[1 10]
  Unit Delay : UnitDelay  SampleTime=1e-6  HasFrameUpgradeWarning=on
  Unit Delay1 : UnitDelay  SampleTime=1e-6  HasFrameUpgradeWarning=on
  Unit Delay2 : UnitDelay  InitialCondition=600  SampleTime=1e-6  HasFrameUpgradeWarning=on
  Unit Delay3 : UnitDelay  SampleTime=1e-6  HasFrameUpgradeWarning=on
  Voltage Sensor : fl_lib/Electrical/Electrical Sensors/Voltage Sensor
  wires:
  Unit Delay2/1 -> "PWM Timing and Waveform Generator (Three-phase, Two-level)"/2
  PS-Simulink Converter6/1 -> Unit Delay2/1
  MATLAB Function/1(optimal_mod_index) -> Sine Wave Generator (Three-Phase)/1
  PS-Simulink Converter4/1 -> Demux1/1
  Unit Delay/1 -> Transfer Fcn/1
  Demux1/4 -> Transfer Fcn1/1
  RMS/1 -> Unit Delay/1
  Constant/1 -> Slider Gain/1
  Constant2/1 -> TPF Function/3(T_amb)
  Demux/2 -> Scope2/2, Simulink-PS Converter2/1
  Slider Gain/1 -> Sine Wave Generator (Three-Phase)/3
  Transfer Fcn/1 -> Math Function/1, TPF Function/1(I_rms)
  Demux/3 -> Scope2/3, Simulink-PS Converter/1
  Transfer Fcn1/1 -> Unit Delay1/1
  Math Function/1 -> Gain/1
  PS-Simulink Converter1/1 -> RMS/1
  Sine Wave Generator (Three-Phase)/2 -> Scope3/1
  Sine Wave Generator (Three-Phase)/1 -> "PWM Timing and Waveform Generator (Three-phase, Two-level)"/1, Scope/1
  Demux/1 -> Scope2/1, Simulink-PS Converter1/1
  Constant1/1 -> Sine Wave Generator (Three-Phase)/2
  Gain/1 -> Integrator/1
  Integrator/1 -> TPF Function/2(T_curr)
  TPF Function/1(derating_cmd) -> Unit Delay3/1
  Unit Delay3/1 -> MATLAB Function/3(current_mod_index)
  Constant3/1 -> Simulink-PS Converter3/1
  PS-Simulink Converter2/1 -> Scope4/2
  PS-Simulink Converter3/1 -> Scope4/1
  PS-Simulink Converter7/1 -> Transfer Fcn3/1
  Transfer Fcn3/1 -> RMS2/1
  PS-Simulink Converter5/1 -> Transfer Fcn2/1
  Transfer Fcn2/1 -> RMS1/1
  RMS1/1 -> Scope1/1
  RMS2/1 -> MATLAB Function/1(accel)
  "PWM Timing and Waveform Generator (Three-phase, Two-level)"/1 -> Scope5/1, Demux/1
  Unit Delay1/1 -> MATLAB Function/2(vibration_rms)
  connections:
  Half-Bridge Driver/RConn2 -- Current Sensor/LConn1 -- "MOSFET (Ideal, Switching)"/RConn2 -- Current Sensor/RConn2 -- "MOSFET (Ideal, Switching)5"/RConn1 -- Induction Machine Squirrel Cage1/RConn2
  DC Voltage Source/LConn1 -- Voltage Sensor/LConn1 -- "MOSFET (Ideal, Switching)2"/RConn1 -- "MOSFET (Ideal, Switching)1"/RConn1 -- "MOSFET (Ideal, Switching)"/RConn1 -- Solver Configuration/RConn1 -- Capacitor2/LConn1 -- Capacitor5/LConn1 -- Capacitor1/LConn1 -- Capacitor4/LConn1 -- Capacitor/LConn1 -- Capacitor3/LConn1
  Induction Machine Squirrel Cage1/RConn5 -- Induction Machine Squirrel Cage1/RConn7 -- Induction Machine Squirrel Cage1/RConn6
  "MOSFET (Ideal, Switching)2"/RConn2 -- "MOSFET (Ideal, Switching)3"/RConn1 -- Half-Bridge Driver3/RConn2 -- Induction Machine Squirrel Cage1/RConn4
  "MOSFET (Ideal, Switching)5"/RConn2 -- Half-Bridge Driver/RConn4 -- Half-Bridge Driver2/RConn4 -- "MOSFET (Ideal, Switching)4"/RConn2 -- Half-Bridge Driver3/RConn4 -- "MOSFET (Ideal, Switching)3"/RConn2 -- Capacitor5/RConn1 -- Capacitor3/RConn1 -- Capacitor2/RConn1 -- Capacitor/RConn1 -- Capacitor4/RConn1 -- Capacitor1/RConn1 -- Voltage Sensor/RConn2 -- Electrical Reference/LConn1 -- DC Voltage Source/RConn1
  "MOSFET (Ideal, Switching)4"/RConn1 -- "MOSFET (Ideal, Switching)1"/RConn2 -- Half-Bridge Driver2/RConn2 -- Induction Machine Squirrel Cage1/RConn3
  Voltage Sensor/RConn1 -- PS-Simulink Converter6/LConn1
  Simulink-PS Converter2/RConn1 -- Half-Bridge Driver2/LConn1
  Half-Bridge Driver/RConn1 -- "MOSFET (Ideal, Switching)"/LConn1
  Simulink-PS Converter/RConn1 -- Half-Bridge Driver/LConn1
  "MOSFET (Ideal, Switching)3"/LConn1 -- Half-Bridge Driver3/RConn3
  Current Sensor/RConn1 -- PS-Simulink Converter1/LConn1
  Half-Bridge Driver/RConn3 -- "MOSFET (Ideal, Switching)5"/LConn1
  "MOSFET (Ideal, Switching)1"/LConn1 -- Half-Bridge Driver2/RConn1
  "MOSFET (Ideal, Switching)4"/LConn1 -- Half-Bridge Driver2/RConn3
  Induction Machine Squirrel Cage1/RConn1 -- PS-Simulink Converter4/LConn1
  Simulink-PS Converter1/RConn1 -- Half-Bridge Driver3/LConn1
  "MOSFET (Ideal, Switching)2"/LConn1 -- Half-Bridge Driver3/RConn1
  Simulink-PS Converter3/RConn1 -- Ideal Torque Source/RConn1
  Ideal Rotational Motion Sensor1/LConn1 -- Inertia1/RConn1 -- Induction Machine Squirrel Cage1/LConn1 -- Rotational Damper/LConn1 -- Inertia1/LConn1 -- Ideal Torque Source/LConn1 -- Ideal Torque Sensor/LConn1
  Rotational Damper/RConn1 -- Mechanical Rotational Reference/LConn1 -- Ideal Torque Source/RConn2 -- Induction Machine Squirrel Cage1/LConn2 -- Ideal Torque Sensor/RConn1
  Ideal Torque Sensor/RConn2 -- PS-Simulink Converter2/LConn1
  Ideal Rotational Motion Sensor1/RConn4 -- PS-Simulink Converter3/LConn1
  Ideal Rotational Motion Sensor1/RConn1 -- Mechanical Rotational Reference1/LConn1
  Ideal Rotational Motion Sensor1/RConn3 -- PS-Simulink Converter5/LConn1
  Ideal Rotational Motion Sensor1/RConn2 -- PS-Simulink Converter7/LConn1

== matlab function VFDnow/TPF Function ==
  settings: updateMethod=DISCRETE
  data: I_rms input; derating_cmd output; T_curr input; T_amb input
function derating_cmd = TPF_Controller(I_rms, T_curr, T_amb)
    persistent I_term;
    if isempty(I_term), I_term = 0; end
    
    % Prediction: Heat gain (I^2) vs Cooling (Delta T)
    % Using a small DT for real-time simulation steps
    DT = 0.001; 
    T_pred = T_curr + ((0.05 * I_rms^2) - (0.01 * (T_curr - T_amb))) * DT;
    
    SAFE_LIMIT = 100.0;
    error = SAFE_LIMIT - T_pred;
    
    % PI Derating Logic
    if error < 0 % We are exceeding or about to exceed the limit
        I_term = I_term + (0.01 * error); % Integral action
        output = 1.0 + (0.05 * error) + I_term; 
    else
        I_term = 0; % Reset when safe
        output = 1.0;
    end
    
    % Clamp between 10% (limp home mode) and 100%
    derating_cmd = max(min(output, 1.0), 0.1);
end

== matlab function VFDnow/MATLAB Function ==
  settings: updateMethod=DISCRETE
  data: accel input; optimal_mod_index output; vibration_rms input; current_mod_index input
function optimal_mod_index = POF_Controller(accel, vibration_rms, current_mod_index)
    % Initialize persistent variables for memory across time steps
    persistent best_voltage state wait_timer
    
    % Step size for optimization
    step_size = 0.01;
    
    % Initialize if first run
    if isempty(best_voltage)
        best_voltage = 1.0; 
        state = 0; 
        wait_timer = 0;
    end
    
    % Constants for Hyperloop Logic
    CRUISE_ACCEL = 0.05; 
    MAX_VIBE = 0.5;
    
    % Logic State Machine
    switch state
        case 0 % MONITORING: If cruising at low accel, start reducing voltage for efficiency
            if abs(accel) < CRUISE_ACCEL
                state = 1; 
            else
                best_voltage = 1.0; 
            end
        case 1 % OPTIMIZING: Reduce voltage until vibration becomes too high
            if vibration_rms > MAX_VIBE
                state = 2; 
            else
                best_voltage = best_voltage - step_size; 
            end
        case 2 % RECOVERY: Increase voltage back to safe levels
            best_voltage = best_voltage + 0.05;
            wait_timer = wait_timer + 1;
            if wait_timer > 100
                wait_timer = 0; 
                state = 0; 
            end
        otherwise
            state = 0; % Safety catch-all
    end
    
    % Final Output: Constrain between 0.4 and 1.0
    % We multiply by current_mod_index to ensure it respects the TPF derating
    % Final Output: Constrain between 0.4 and 1.0
    % Multiply by current_mod_index to ensure it respects the TPF derating
    temp_out = best_voltage * current_mod_index; 
    optimal_mod_index = max(min(temp_out, 1.0), 0.4);
end
